simulink model "BasePerTracing_2023a"  (R2023a)
settings: Solver=FixedStepDiscrete  StartTime=0.0  StopTime=Inf  RelTol=1e-3  EnableMultiTasking=on
InitFcn:
  | mcb_pmsm_foc_qep_f28379d_data;
values from neighbouring files (symbols this model uses):
  ADCCount = ADCResolution-1    (= 4095)    [parameters.m]
  GainVsense = 4.99/(62+4.99)    (= 0.0744887296611)    [parameters.m]
  J = Jdc + Jbl    (= 7.32e-05)    [parameters.m]
  Km = 0.11    [parameters.m]
  Kpi = L/taui    (= 4.1)    [parameters.m]
  Kpv = J/(tauv*Km)    (= 0.0665454545455)    [parameters.m]
  OffsetADCINC4 = 2296    [parameters.m]
  PulseNumber = 2048*4    (= 8192)    [parameters.m]
  RadiantsPerCount = 2*pi/(PulseNumber-1)    (= 0.00076708403213)    [parameters.m]
  TaoFilterOffsetCurrent = 1    [parameters.m]
  TaoFilterOmega = 0.002    [parameters.m]
  Tii = L/R    (= 0.00128125)    [parameters.m]
  Tiv = Taom    (= 0.085)    [parameters.m]
  TSample = 0.0001    [parameters.m]
  VrefADC = 3    [parameters.m]
undefined symbols (not defined in the file or in its folder): dataType, Down, GPTRIP1SEL, GPTRIP2SEL, TZ1, TZ2, Up
libraries: c2802xlib x9, simulink x6, c280xlib x4, c2837xDlib x3, c2000lib x1, svdutilitieslib x1
(part 2 of 2)

== matlab function BasePerTracing_2023a/Current Control/ENCODER/MATLAB Function ==
  data: Ts input; out output; Tao input; In input
function out  = LowPassFilter(  Ts ,Tao, In)

persistent OutPrecedente
if isempty( OutPrecedente )
    OutPrecedente = 0 ;
end
    %Filtro passa basso discretizzato con il metodo delle differenze
    %all'indietro
    
    a=Ts/(Ts+Tao);
    b=Tao/(Ts+Tao);
    
    out=a*In+OutPrecedente*b;
   
    OutPrecedente = out;
   
end
